simulink model "Validation_TopOil"  (R2025a)
settings: Solver=VariableStepAuto  StartTime=0.0  StopTime=StopTime_s  MaxStep=3600  RelTol=1e-3
values from neighbouring files (symbols this model uses):
  B = 7.5    [half_year_bias.m]    (also in step4_inputs.mat; step4_prepare_inputs.m; step5_fit_formA_vs_formB.m; step5_results.mat)
  n = 0.8    [half_year_bias.m]    (also in step2_results.mat; step2_run_topoil_model.m; step3_fit_parameters.m; step3_results.mat)
  THETA_O_R = 64.7691731483    [step4_inputs.mat]    (also in step4_prepare_inputs.m = p_cal(1))
  Theta_TO_0 = 7.6325    [step4_inputs.mat]    (also in step4_prepare_inputs.m = TOv(1))
  Tt_O = 480.460516355    [step4_inputs.mat]    (also in step4_prepare_inputs.m = p_cal(2) * 60)
settings Model: Creator=Mahammad  LastModifiedBy=Mahammad

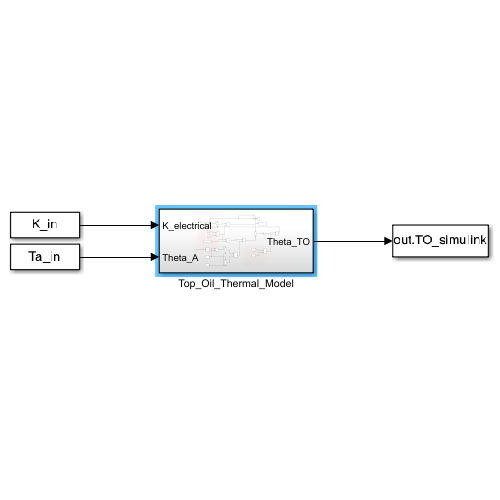
[thumbnail: Simulink's stored preview of the top-level diagram]
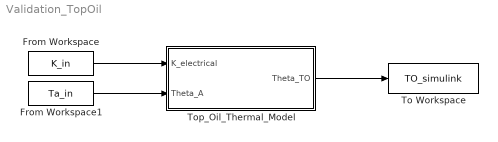
== system Validation_TopOil ==
  From Workspace : FromWorkspace  VariableName=K_in  Interpolate=off  OutputAfterFinalValue=Holding final value
  From Workspace1 : FromWorkspace  VariableName=Ta_in  Interpolate=off  OutputAfterFinalValue=Holding final value
  To Workspace : ToWorkspace  VariableName=TO_simulink  SaveFormat=Timeseries  SampleTime=-1
  Top_Oil_Thermal_Model : Subsystem
  wires:
  From Workspace/1 -> Top_Oil_Thermal_Model/1(K_electrical)
  Top_Oil_Thermal_Model/1(Theta_TO) -> To Workspace/1
  From Workspace1/1 -> Top_Oil_Thermal_Model/2(Theta_A)

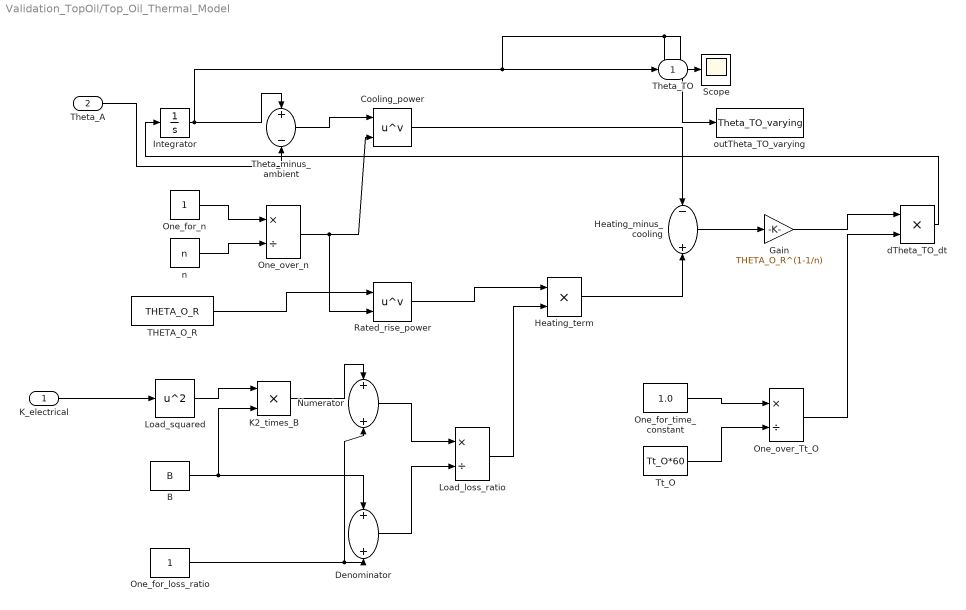
== system Validation_TopOil/Top_Oil_Thermal_Model ==
  K_electrical : Inport
  Theta_A : Inport  Port=2
  B : Constant  Value=B
  Cooling_power : Math  Operator=pow  SignedPower=on
  Denominator : Sum
  Gain : Gain  Gain=THETA_O_R^(1-1/n)
  Heating_minus_cooling : Sum  Inputs=-+
  Heating_term : Product  Inputs=**
  Integrator : Integrator  InitialCondition=Theta_TO_0
  K2_times_B : Product  Inputs=**
  Load_loss_ratio : Product  Inputs=*/
  Load_squared : Math  Operator=square
  Numerator : Sum
  One_for_loss_ratio : Constant
  One_for_n : Constant
  One_for_time_constant : Constant  Value=1.0
  One_over_Tt_O : Product  Inputs=*/
  One_over_n : Product  Inputs=*/
  Rated_rise_power : Math  Operator=pow  SignedPower=on
  Scope : Scope
      settings: ActiveDisplayYMinimum=-1  ActiveDisplayYMaximum=1
  THETA_O_R : Constant  Value=THETA_O_R
  Theta_minus_ambient : Sum  Inputs=+-
  Tt_O : Constant  Value=Tt_O*60
  dTheta_TO_dt : Product  Inputs=**
  n : Constant  Value=n
  outTheta_TO_varying : ToWorkspace  VariableName=Theta_TO_varying  SaveFormat=Structure With Time  SampleTime=-1
  Theta_TO : Outport
  wires:
  Integrator/1 -> Theta_TO/1, outTheta_TO_varying/1, Scope/1, Theta_minus_ambient/1
  dTheta_TO_dt/1 -> Integrator/1
  B/1 -> K2_times_B/2, Denominator/1
  Theta_A/1 -> Theta_minus_ambient/2
  Cooling_power/1 -> Heating_minus_cooling/1
  One_over_n/1 -> Cooling_power/2, Rated_rise_power/2
  Load_squared/1 -> K2_times_B/1
  Tt_O/1 -> One_over_Tt_O/2
  Denominator/1 -> Load_loss_ratio/2
  One_for_time_constant/1 -> One_over_Tt_O/1
  Heating_term/1 -> Heating_minus_cooling/2
  One_for_loss_ratio/1 -> Numerator/2, Denominator/2
  K2_times_B/1 -> Numerator/1
  Theta_minus_ambient/1 -> Cooling_power/1
  Load_loss_ratio/1 -> Heating_term/2
  Rated_rise_power/1 -> Heating_term/1
  Numerator/1 -> Load_loss_ratio/1
  THETA_O_R/1 -> Rated_rise_power/1
  One_for_n/1 -> One_over_n/1
  n/1 -> One_over_n/2
  K_electrical/1 -> Load_squared/1
  One_over_Tt_O/1 -> dTheta_TO_dt/2
  Heating_minus_cooling/1 -> Gain/1
  Gain/1 -> dTheta_TO_dt/1
